simulink model "Sim2Real_variant_subsystem"  (R2025b)
settings: Solver=FixedStepDiscrete  StartTime=0.0  StopTime=inf  FixedStep=Ts_1ms  MaxStep=0.002  RelTol=1e-3
InitFcn:
  | modelFile = get_param(bdroot,'FileName');
  | if isempty(modelFile)
  |     error('The model must be saved before running InitFcn.');
  | end
  | 
  | % Folder where the .slx model is located
  | modelFolder = fileparts(char(modelFile));
  | 
  | % Find the parent folder named "resources" by going upwards
  | currentFolder  = modelFolder;
  | materialFolder = '';
  | 
  | while true
  |     [parentFolder, currentName] = fileparts(currentFolder);
  | 
  |     if strcmpi(currentName, 'resources')
  |         materialFolder = currentFolder;
  |         break;
  |     end
  | 
  |     if strcmp(parentFolder, currentFolder)
  |         error('Could not find a parent folder named "resources" starting from: %s', modelFolder);
  |     end
  | 
  |     currentFolder = parentFolder;
  | end
  | 
  | % Search recursively for the MuJoCo XML inside "material"
  | xmlSearch = dir(fullfile(materialFolder, '**', 'unitree_G1.xml'));
  | 
  | if isempty(xmlSearch)
  |     error('MuJoCo XML file not found inside material folder: %s', materialFolder);
  | elseif numel(xmlSearch) > 1
  |     error('Multiple unitree_G1.xml files found inside material folder. Leave only one valid XML.');
  | end
  | 
  | mujocoFolder = xmlSearch(1).folder;
  | xmlFullPath  = fullfile(xmlSearch(1).folder, xmlSearch(1).name);
  | 
  | % Save in base workspace in case you want to inspect them
  | assignin('base','modelFolder',modelFolder);
  | assignin('base','materialFolder',materialFolder);
  | assignin('base','mujocoFolder',mujocoFolder);
  | assignin('base','xmlFullPath',xmlFullPath);
  | 
  | % Final existence check
  | if exist(xmlFullPath,'file') ~= 2
  |     error('MuJoCo XML file not found: %s', xmlFullPath);
  | end
  | 
  | % Add the XML folder to the path so WHICH can find it
  | addpath(mujocoFolder, '-begin');
  | rehash path;
  | 
  | % Run launcher from the same folder as the model
  | launcherFile = fullfile(modelFolder, 'launcher.mlx');
  | if exist(launcherFile,'file') == 2
  |     run(launcherFile);
  | else
  |     error('Launcher file not found: %s', launcherFile);
  | end
  | 
  | % RUN_MODE:
  | if evalin('base', "exist('RUN_MODE','var')")
  |     tmp = evalin('base','RUN_MODE');
  |     if isa(tmp,'Simulink.Parameter')
  |         RUN_MODE = tmp;
  |     else
  |         RUN_MODE = Simulink.Parameter(tmp);
  |         RUN_MODE.CoderInfo.StorageClass = 'SimulinkGlobal';
  |         assignin('base','RUN_MODE',RUN_MODE);
  |     end
  | else
  |     RUN_MODE = Simulink.Parameter(0);
  |     RUN_MODE.CoderInfo.StorageClass = 'SimulinkGlobal';
  |     assignin('base','RUN_MODE',RUN_MODE);
  | end
StopFcn:
  | drawnow; pause(0.05);
  | 
  | % Stop figures
  | tags = {'G1_IMUState','G1_MotorState'};
  | for k = 1:numel(tags)
  |     delete(findall(0,'Type','uifigure','Tag',tags{k}));
  |     delete(findall(0,'Type','figure' , 'Tag',tags{k}));
  | end
undefined symbols (not defined in the file): crc, mode_machine, mode_pr, motor_cmd, reserve, Ts_1ms
libraries: ros2lib x3, mjLib x1
(part 1 of 2)
settings Model: Creator=vmano  LastModifiedBy=leffe
settings OptimizationCC: ReuseModelBlockBuffer=off
settings ModelReferenceCC: EnableRefExpFcnMdlSchedulingChecks=on
settings SFSimCC: SimTargetLang=C++  SimDLTargetLibrary=mkl-dnn
settings RTWCC: GPUComputeCapability=3.5

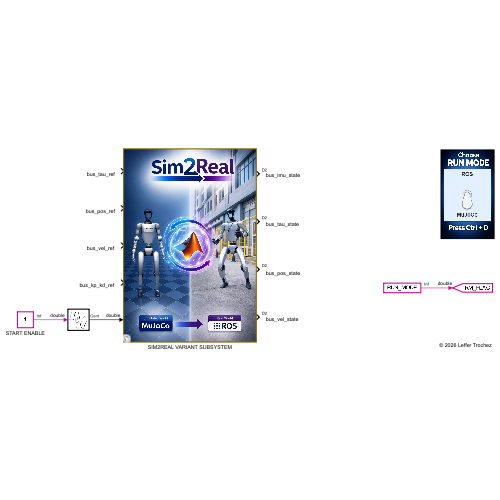
[thumbnail: Simulink's stored preview of the top-level diagram]
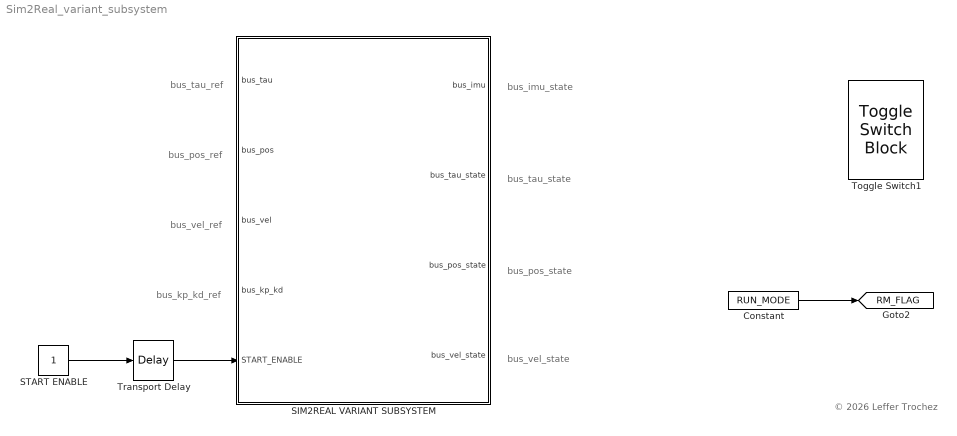
== system Sim2Real_variant_subsystem ==
  note: bus_tau_ref
  note: © 2026 Leffer Trochez
  note: bus_pos_ref
  note: bus_vel_ref
  note: bus_kp_kd_ref
  note: bus_imu_state
  note: bus_tau_state
  note: bus_pos_state
  note: bus_vel_state
  Constant : Constant  Value=RUN_MODE
  SIM2REAL VARIANT SUBSYSTEM : Subsystem  Variant=on  EmptyChoice=on
      mask Display: image('Sim2RealLogo2.png');
  START ENABLE : Constant
  Toggle Switch1 : ToggleSwitchBlock  LabelPosition=Hide
  Transport Delay : TransportDelay  DelayTime=2
  tag scope: RM_FLAG=global
  wires:
  START ENABLE/1 -> Transport Delay/1
  Constant/1 -> [RM_FLAG]
  Transport Delay/1 -> SIM2REAL VARIANT SUBSYSTEM/5(START_ENABLE)

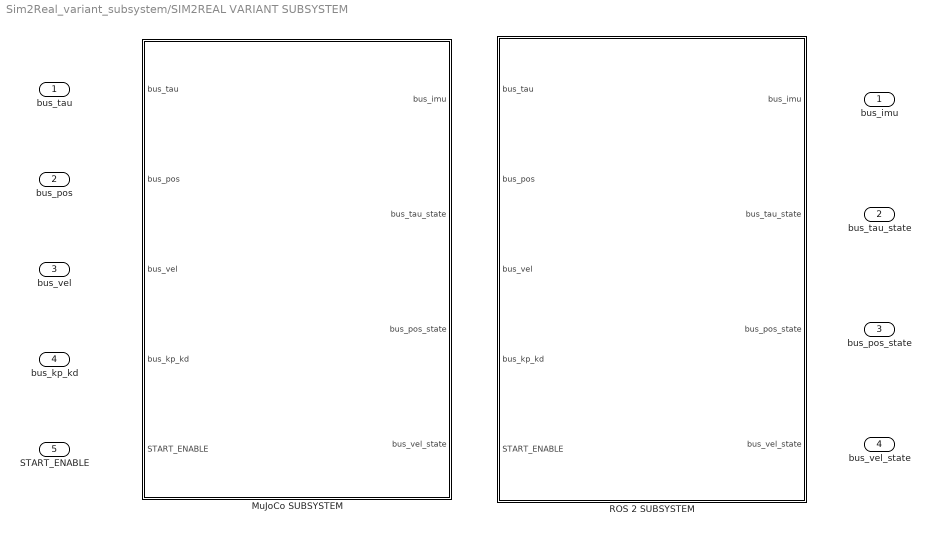
== system Sim2Real_variant_subsystem/SIM2REAL VARIANT SUBSYSTEM ==
  bus_tau : Inport  OutDataTypeStr=Bus: bus_tau_ref
  bus_pos : Inport  Port=2  OutDataTypeStr=Bus: bus_pos_ref
  bus_vel : Inport  Port=3  OutDataTypeStr=Bus: bus_vel_ref
  bus_kp_kd : Inport  Port=4  OutDataTypeStr=Bus: bus_kp_kd_dyn
  START_ENABLE : Inport  Port=5
  MuJoCo SUBSYSTEM : Subsystem  VariantControl=RUN_MODE == 0
      mask Display: image('MuJoCo G1.png');
  ROS 2 SUBSYSTEM : Subsystem  VariantControl=RUN_MODE == 1
      mask Display: image('Real G1.png');
  bus_imu : Outport  OutDataTypeStr=Bus: bus_imu
  bus_tau_state : Outport  Port=2  OutDataTypeStr=Bus: bus_tau_state
  bus_pos_state : Outport  Port=3  OutDataTypeStr=Bus: bus_pos_state
  bus_vel_state : Outport  Port=4  OutDataTypeStr=Bus: bus_vel_state

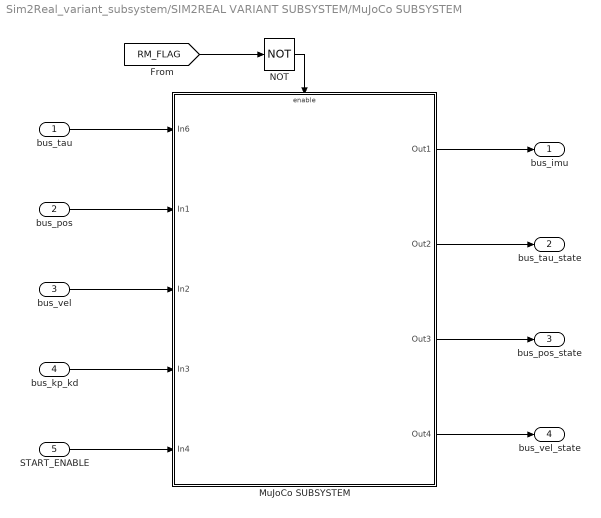
== system Sim2Real_variant_subsystem/SIM2REAL VARIANT SUBSYSTEM/MuJoCo SUBSYSTEM ==
  bus_tau : Inport  OutDataTypeStr=Bus: bus_tau_ref
  bus_pos : Inport  Port=2  OutDataTypeStr=Bus: bus_pos_ref
  bus_vel : Inport  Port=3  OutDataTypeStr=Bus: bus_vel_ref
  bus_kp_kd : Inport  Port=4  OutDataTypeStr=Bus: bus_kp_kd_dyn
  START_ENABLE : Inport  Port=5
  MuJoCo SUBSYSTEM : Subsystem  TreatAsAtomicUnit=on
      mask Display: image('MuJoCo G1.png');
  NOT : Logic  Operator=NOT  IconShape=distinctive  AllPortsSameDT=off  OutDataTypeStr=boolean
  bus_imu : Outport  OutDataTypeStr=Bus: bus_imu
  bus_tau_state : Outport  Port=2  OutDataTypeStr=Bus: bus_tau_state
  bus_pos_state : Outport  Port=3  OutDataTypeStr=Bus: bus_pos_state
  bus_vel_state : Outport  Port=4  OutDataTypeStr=Bus: bus_vel_state
  wires:
  [RM_FLAG] -> NOT/1
  NOT/1 -> MuJoCo SUBSYSTEM/Enable
  bus_tau/1 -> MuJoCo SUBSYSTEM/1(In6)
  bus_pos/1 -> MuJoCo SUBSYSTEM/2(In1)
  bus_vel/1 -> MuJoCo SUBSYSTEM/3(In2)
  bus_kp_kd/1 -> MuJoCo SUBSYSTEM/4(In3)
  START_ENABLE/1 -> MuJoCo SUBSYSTEM/5(In4)
  MuJoCo SUBSYSTEM/1(Out1) -> bus_imu/1
  MuJoCo SUBSYSTEM/2(Out2) -> bus_tau_state/1
  MuJoCo SUBSYSTEM/3(Out3) -> bus_pos_state/1
  MuJoCo SUBSYSTEM/4(Out4) -> bus_vel_state/1

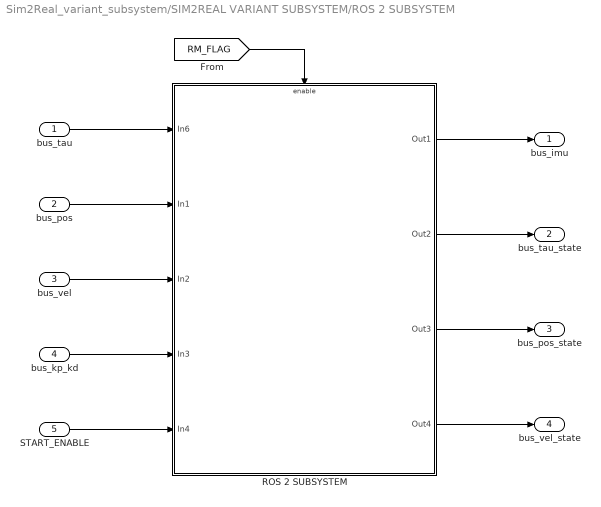
== system Sim2Real_variant_subsystem/SIM2REAL VARIANT SUBSYSTEM/ROS 2 SUBSYSTEM ==
  bus_tau : Inport  OutDataTypeStr=Bus: bus_tau_ref
  bus_pos : Inport  Port=2  OutDataTypeStr=Bus: bus_pos_ref
  bus_vel : Inport  Port=3  OutDataTypeStr=Bus: bus_vel_ref
  bus_kp_kd : Inport  Port=4  OutDataTypeStr=Bus: bus_kp_kd_dyn
  START_ENABLE : Inport  Port=5
  ROS 2 SUBSYSTEM : Subsystem  TreatAsAtomicUnit=on
      mask Display: image('Real G1.png');
  bus_imu : Outport  OutDataTypeStr=Bus: bus_imu
  bus_tau_state : Outport  Port=2  OutDataTypeStr=Bus: bus_tau_state
  bus_pos_state : Outport  Port=3  OutDataTypeStr=Bus: bus_pos_state
  bus_vel_state : Outport  Port=4  OutDataTypeStr=Bus: bus_vel_state
  wires:
  bus_tau/1 -> ROS 2 SUBSYSTEM/1(In6)
  bus_kp_kd/1 -> ROS 2 SUBSYSTEM/4(In3)
  bus_vel/1 -> ROS 2 SUBSYSTEM/3(In2)
  START_ENABLE/1 -> ROS 2 SUBSYSTEM/5(In4)
  bus_pos/1 -> ROS 2 SUBSYSTEM/2(In1)
  ROS 2 SUBSYSTEM/3(Out3) -> bus_pos_state/1
  ROS 2 SUBSYSTEM/2(Out2) -> bus_tau_state/1
  ROS 2 SUBSYSTEM/1(Out1) -> bus_imu/1
  ROS 2 SUBSYSTEM/4(Out4) -> bus_vel_state/1
  [RM_FLAG] -> ROS 2 SUBSYSTEM/Enable

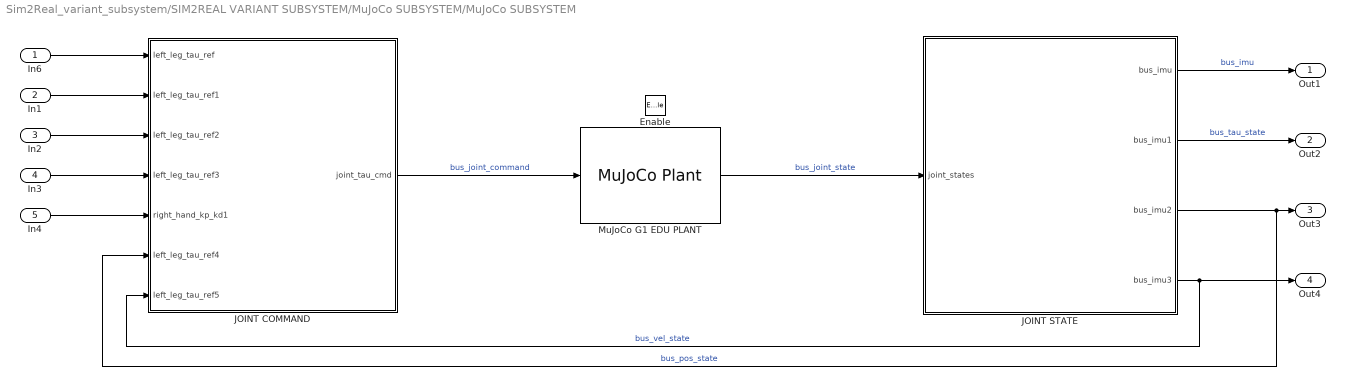
== system Sim2Real_variant_subsystem/SIM2REAL VARIANT SUBSYSTEM/MuJoCo SUBSYSTEM/MuJoCo SUBSYSTEM ==
  In6 : Inport  OutDataTypeStr=Bus: bus_tau_ref
  In1 : Inport  Port=2  OutDataTypeStr=Bus: bus_pos_ref
  In2 : Inport  Port=3  OutDataTypeStr=Bus: bus_vel_ref
  In3 : Inport  Port=4  OutDataTypeStr=Bus: bus_kp_kd_dyn
  In4 : Inport  Port=5
  Enable : EnablePort
  JOINT COMMAND : Subsystem
      mask Display: image('1.png');
  JOINT STATE : Subsystem
      mask Display: image('2.png');
  MuJoCo G1 EDU PLANT : mjLib/MuJoCo Plant  controlBus=[]  sensorBus=mj_bus_sensor_7979902499018342666  controlLength=[]  sensorLength=[]  rgbLength=[]  depthLength=[]  sampleTime=0.002  xmlFileRel=unitree_G1.xml  xmlFile=C:\Users\leffe\OneDrive - Universidad de los andes\GIAP research group\Conferences\ICRA 2026 - poster Sim2Real G1\resources\MuJoCo files\unitree_G1.xml  renderingType=Global  vsync=off  visualFPS=FPS_MuJoCo  zoomLevel=1  znear=0.032  zfar=160  cameraSampleTime=Ts_1ms  rgbOutOption=on  depthOutOption=off  controlInterfaceType=Bus
      settings: SourceProductName=MuJoCo Simulator
  Out1 : Outport  OutDataTypeStr=Bus: bus_imu
  Out2 : Outport  Port=2  OutDataTypeStr=Bus: bus_tau_state
  Out3 : Outport  Port=3  OutDataTypeStr=Bus: bus_pos_state
  Out4 : Outport  Port=4  OutDataTypeStr=Bus: bus_vel_state
  wires:
  JOINT COMMAND/1(joint_tau_cmd) -> MuJoCo G1 EDU PLANT/1  "bus_joint_command"
  MuJoCo G1 EDU PLANT/1 -> JOINT STATE/1(joint_states)  "bus_joint_state"
  In6/1 -> JOINT COMMAND/1(left_leg_tau_ref)
  In1/1 -> JOINT COMMAND/2(left_leg_tau_ref1)
  In2/1 -> JOINT COMMAND/3(left_leg_tau_ref2)
  In3/1 -> JOINT COMMAND/4(left_leg_tau_ref3)
  In4/1 -> JOINT COMMAND/5(right_hand_kp_kd1)
  JOINT STATE/2(bus_imu1) -> Out2/1  "bus_tau_state"
  JOINT STATE/3(bus_imu2) -> JOINT COMMAND/6(left_leg_tau_ref4), Out3/1  "bus_pos_state"
  JOINT STATE/4(bus_imu3) -> Out4/1, JOINT COMMAND/7(left_leg_tau_ref5)  "bus_vel_state"
  JOINT STATE/1(bus_imu) -> Out1/1  "bus_imu"

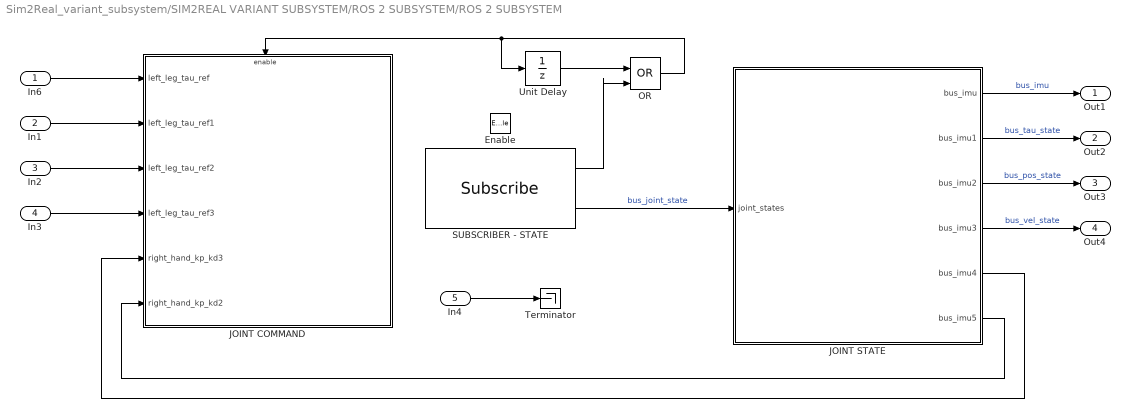
== system Sim2Real_variant_subsystem/SIM2REAL VARIANT SUBSYSTEM/ROS 2 SUBSYSTEM/ROS 2 SUBSYSTEM ==
  In6 : Inport  OutDataTypeStr=Bus: bus_tau_ref
  In1 : Inport  Port=2  OutDataTypeStr=Bus: bus_pos_ref
  In2 : Inport  Port=3  OutDataTypeStr=Bus: bus_vel_ref
  In3 : Inport  Port=4  OutDataTypeStr=Bus: bus_kp_kd_dyn
  In4 : Inport  Port=5
  Enable : EnablePort
  JOINT COMMAND : Subsystem  TreatAsAtomicUnit=on
      mask Display: image('8.png');
  JOINT STATE : Subsystem
      mask Display: image('9.png');
  OR : Logic  Operator=OR  IconShape=distinctive  AllPortsSameDT=off  OutDataTypeStr=boolean
  SUBSCRIBER - STATE : ros2lib/Subscribe  topicSource=Specify your own  topic=/lowstate  messageType=unitree_hg/LowState  sampleTime=Ts_1ms  QOSHistory=Keep last  QOSDepth=10  QOSReliability=Reliable  QOSDurability=Volatile  QOSDeadline=Inf  QOSLifespan=Inf  QOSLiveliness=Automatic  QOSLeaseDuration=Inf  QOSAvoidROSNamespaceConventions=off
  Terminator : Terminator
  Unit Delay : UnitDelay  SampleTime=0.002  HasFrameUpgradeWarning=on
  Out1 : Outport  OutDataTypeStr=Bus: bus_imu
  Out2 : Outport  Port=2  OutDataTypeStr=Bus: bus_tau_state
  Out3 : Outport  Port=3  OutDataTypeStr=Bus: bus_pos_state
  Out4 : Outport  Port=4  OutDataTypeStr=Bus: bus_vel_state
  wires:
  SUBSCRIBER - STATE/2 -> JOINT STATE/1(joint_states)  "bus_joint_state"
  SUBSCRIBER - STATE/1 -> OR/2
  OR/1 -> JOINT COMMAND/Enable, Unit Delay/1
  Unit Delay/1 -> OR/1
  JOINT STATE/6(bus_imu5) -> JOINT COMMAND/6(right_hand_kp_kd2)
  In2/1 -> JOINT COMMAND/3(left_leg_tau_ref2)
  In3/1 -> JOINT COMMAND/4(left_leg_tau_ref3)
  In4/1 -> Terminator/1
  In1/1 -> JOINT COMMAND/2(left_leg_tau_ref1)
  In6/1 -> JOINT COMMAND/1(left_leg_tau_ref)
  JOINT STATE/4(bus_imu3) -> Out4/1  "bus_vel_state"
  JOINT STATE/3(bus_imu2) -> Out3/1  "bus_pos_state"
  JOINT STATE/2(bus_imu1) -> Out2/1  "bus_tau_state"
  JOINT STATE/1(bus_imu) -> Out1/1  "bus_imu"
  JOINT STATE/5(bus_imu4) -> JOINT COMMAND/5(right_hand_kp_kd3)

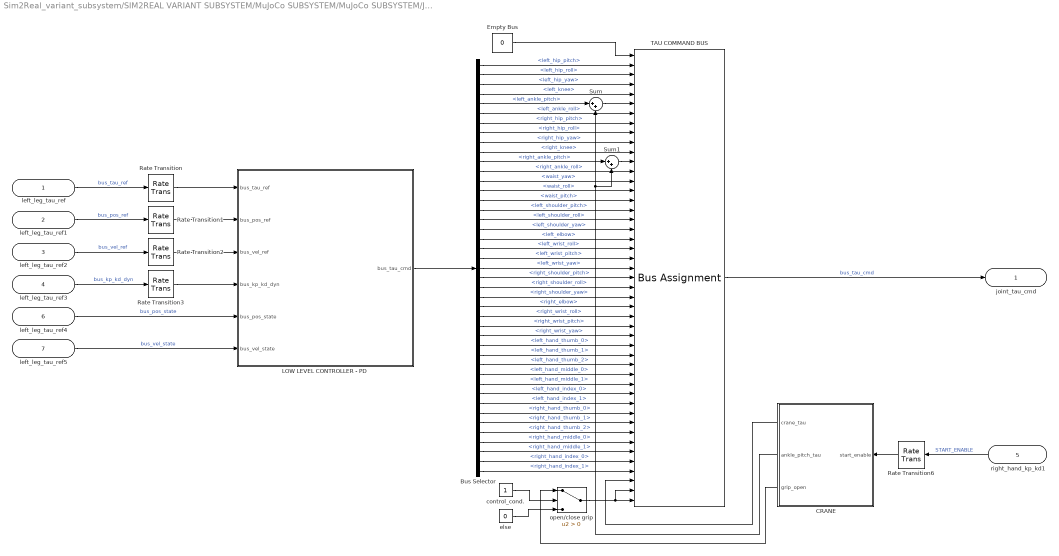
== system Sim2Real_variant_subsystem/SIM2REAL VARIANT SUBSYSTEM/MuJoCo SUBSYSTEM/MuJoCo SUBSYSTEM/JOINT COMMAND ==
  left_leg_tau_ref : Inport  OutDataTypeStr=Bus: bus_tau_ref
  left_leg_tau_ref1 : Inport  Port=2  OutDataTypeStr=Bus: bus_pos_ref
  left_leg_tau_ref2 : Inport  Port=3  OutDataTypeStr=Bus: bus_vel_ref
  left_leg_tau_ref3 : Inport  Port=4  OutDataTypeStr=Bus: bus_kp_kd_dyn
  right_hand_kp_kd1 : Inport  Port=5
  left_leg_tau_ref4 : Inport  Port=6  OutDataTypeStr=Bus: bus_pos_state
  left_leg_tau_ref5 : Inport  Port=7  OutDataTypeStr=Bus: bus_vel_state
  Bus Selector : BusSelector  OutputSignals=left_hip_pitch,left_hip_roll,left_hip_yaw,left_knee,left_ankle_pitch,left_ankle_roll,right_hip_pitch,right_hip_roll,right_hip_yaw,right_knee,right_ankle_pitch,right_ankle_roll,waist_yaw,waist_roll,waist_pitch,left_shoulder_pitch,left_shoulder_roll,left_shoulder_yaw,left_elbow,left_wrist_roll,left_wrist_pitch,left_wrist_yaw,right_shoulder_pitch,right_shoulder_roll,right_shoulder_yaw,right_elbow,right_wrist_roll,right_wrist_pitch,right_wrist_yaw,left_hand_thumb_0,left_hand_thumb_1,left_hand_thumb_2,left_hand_middle_0,left_hand_middle_1,left_hand_index_0,left_hand_index_1,right_hand_thumb_0,right_hand_thumb_1,right_hand_thumb_2,right_hand_middle_0,right_hand_middle_1,right_hand_index_0,right_hand_index_1
  CRANE : MATLAB Function  TreatAsAtomicUnit=on
  Empty Bus : Constant  Value=0  OutDataTypeStr=Bus: mj_bus_input_303657145477151593  LockScale=on
  LOW LEVEL CONTROLLER - PD : MATLAB Function  TreatAsAtomicUnit=on
  Rate Transition{,1..3,6} (5 alike) : RateTransition  OutPortSampleTime=Ts_1ms
  Sum : Sum  Inputs=|++
  Sum1 : Sum  Inputs=|++
  TAU COMMAND BUS : BusAssignment  AssignedSignals=left_hip_pitch,left_hip_roll,left_hip_yaw,left_knee,left_ankle_pitch,left_ankle_roll,right_hip_pitch,right_hip_roll,right_hip_yaw,right_knee,right_ankle_pitch,right_ankle_roll,waist_yaw,waist_roll,waist_pitch,left_shoulder_pitch,left_shoulder_roll,left_shoulder_yaw,left_elbow,left_wrist_roll,left_wrist_pitch,left_wrist_yaw,right_shoulder_pitch,right_shoulder_roll,right_shoulder_yaw,right_elbow,right_wrist_roll,right_wrist_pitch,right_wrist_yaw,left_hand_thumb_0,left_hand_thumb_1,left_hand_thumb_2,left_hand_middle_0,left_hand_middle_1,left_hand_index_0,left_hand_index_1,right_hand_thumb_0,right_hand_thumb_1,right_hand_thumb_2,right_hand_middle_0,right_hand_middle_1,right_hand_index_0,right_hand_index_1,crane_tau,grip_open_R,grip_open_L
  control_cond. : Constant
  else : Constant  Value=0
  open/close grip : Switch  Criteria=u2 > Threshold  SaturateOnIntegerOverflow=off  InputSameDT=off
  joint_tau_cmd : Outport  OutDataTypeStr=Bus: mj_bus_input_303657145477151593
  wires:
  Sum1/1 -> TAU COMMAND BUS/12
  Empty Bus/1 -> TAU COMMAND BUS/1
  CRANE/2(ankle_pitch_tau) -> Sum1/2, Sum/2
  Sum/1 -> TAU COMMAND BUS/6
  CRANE/3(grip_open) -> open/close grip/1
  right_hand_kp_kd1/1 -> Rate Transition6/1  "START_ENABLE"
  TAU COMMAND BUS/1 -> joint_tau_cmd/1  "bus_tau_cmd"
  left_leg_tau_ref/1 -> Rate Transition/1  "bus_tau_ref"
  left_leg_tau_ref1/1 -> Rate Transition1/1  "bus_pos_ref"
  left_leg_tau_ref2/1 -> Rate Transition2/1  "bus_vel_ref"
  left_leg_tau_ref3/1 -> Rate Transition3/1  "bus_kp_kd_dyn"
  left_leg_tau_ref4/1 -> LOW LEVEL CONTROLLER - PD/5(bus_pos_state)  "bus_pos_state"
  left_leg_tau_ref5/1 -> LOW LEVEL CONTROLLER - PD/6(bus_vel_state)  "bus_vel_state"
  CRANE/1(crane_tau) -> TAU COMMAND BUS/45
  Rate Transition/1 -> LOW LEVEL CONTROLLER - PD/1(bus_tau_ref)
  Rate Transition1/1 -> LOW LEVEL CONTROLLER - PD/2(bus_pos_ref)
  Rate Transition2/1 -> LOW LEVEL CONTROLLER - PD/3(bus_vel_ref)
  Rate Transition3/1 -> LOW LEVEL CONTROLLER - PD/4(bus_kp_kd_dyn)
  Rate Transition6/1 -> CRANE/1(start_enable)
  LOW LEVEL CONTROLLER - PD/1(bus_tau_cmd) -> Bus Selector/1
  Bus Selector/11 -> Sum1/1  "<right_ankle_pitch>"
  Bus Selector/5 -> Sum/1  "<left_ankle_pitch>"
  Bus Selector/1 -> TAU COMMAND BUS/2  "<left_hip_pitch>"
  Bus Selector/2 -> TAU COMMAND BUS/3  "<left_hip_roll>"
  Bus Selector/3 -> TAU COMMAND BUS/4  "<left_hip_yaw>"
  Bus Selector/4 -> TAU COMMAND BUS/5  "<left_knee>"
  Bus Selector/6 -> TAU COMMAND BUS/7  "<left_ankle_roll>"
  Bus Selector/7 -> TAU COMMAND BUS/8  "<right_hip_pitch>"
  Bus Selector/8 -> TAU COMMAND BUS/9  "<right_hip_roll>"
  Bus Selector/9 -> TAU COMMAND BUS/10  "<right_hip_yaw>"
  Bus Selector/10 -> TAU COMMAND BUS/11  "<right_knee>"
  Bus Selector/12 -> TAU COMMAND BUS/13  "<right_ankle_roll>"
  Bus Selector/13 -> TAU COMMAND BUS/14  "<waist_yaw>"
  Bus Selector/14 -> TAU COMMAND BUS/15  "<waist_roll>"
  Bus Selector/15 -> TAU COMMAND BUS/16  "<waist_pitch>"
  Bus Selector/16 -> TAU COMMAND BUS/17  "<left_shoulder_pitch>"
  Bus Selector/17 -> TAU COMMAND BUS/18  "<left_shoulder_roll>"
  Bus Selector/18 -> TAU COMMAND BUS/19  "<left_shoulder_yaw>"
  Bus Selector/19 -> TAU COMMAND BUS/20  "<left_elbow>"
  Bus Selector/20 -> TAU COMMAND BUS/21  "<left_wrist_roll>"
  Bus Selector/21 -> TAU COMMAND BUS/22  "<left_wrist_pitch>"
  Bus Selector/22 -> TAU COMMAND BUS/23  "<left_wrist_yaw>"
  Bus Selector/23 -> TAU COMMAND BUS/24  "<right_shoulder_pitch>"
  Bus Selector/24 -> TAU COMMAND BUS/25  "<right_shoulder_roll>"
  Bus Selector/25 -> TAU COMMAND BUS/26  "<right_shoulder_yaw>"
  Bus Selector/26 -> TAU COMMAND BUS/27  "<right_elbow>"
  Bus Selector/27 -> TAU COMMAND BUS/28  "<right_wrist_roll>"
  Bus Selector/28 -> TAU COMMAND BUS/29  "<right_wrist_pitch>"
  Bus Selector/29 -> TAU COMMAND BUS/30  "<right_wrist_yaw>"
  Bus Selector/30 -> TAU COMMAND BUS/31  "<left_hand_thumb_0>"
  Bus Selector/31 -> TAU COMMAND BUS/32  "<left_hand_thumb_1>"
  Bus Selector/32 -> TAU COMMAND BUS/33  "<left_hand_thumb_2>"
  Bus Selector/33 -> TAU COMMAND BUS/34  "<left_hand_middle_0>"
  Bus Selector/34 -> TAU COMMAND BUS/35  "<left_hand_middle_1>"
  Bus Selector/35 -> TAU COMMAND BUS/36  "<left_hand_index_0>"
  Bus Selector/36 -> TAU COMMAND BUS/37  "<left_hand_index_1>"
  Bus Selector/37 -> TAU COMMAND BUS/38  "<right_hand_thumb_0>"
  Bus Selector/38 -> TAU COMMAND BUS/39  "<right_hand_thumb_1>"
  Bus Selector/39 -> TAU COMMAND BUS/40  "<right_hand_thumb_2>"
  Bus Selector/40 -> TAU COMMAND BUS/41  "<right_hand_middle_0>"
  Bus Selector/41 -> TAU COMMAND BUS/42  "<right_hand_middle_1>"
  Bus Selector/42 -> TAU COMMAND BUS/43  "<right_hand_index_0>"
  Bus Selector/43 -> TAU COMMAND BUS/44  "<right_hand_index_1>"
  control_cond./1 -> open/close grip/2
  else/1 -> open/close grip/3
  open/close grip/1 -> TAU COMMAND BUS/47, TAU COMMAND BUS/46

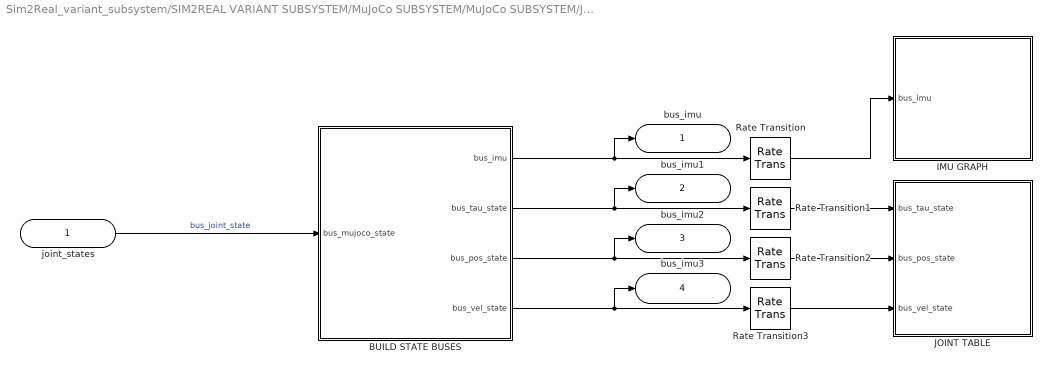
== system Sim2Real_variant_subsystem/SIM2REAL VARIANT SUBSYSTEM/MuJoCo SUBSYSTEM/MuJoCo SUBSYSTEM/JOINT STATE ==
  joint_states : Inport  OutDataTypeStr=Bus: mj_bus_sensor_13323796724550544295
  BUILD STATE BUSES : MATLAB Function  TreatAsAtomicUnit=on
  IMU GRAPH : MATLAB Function  TreatAsAtomicUnit=on
  JOINT TABLE : MATLAB Function  TreatAsAtomicUnit=on
  Rate Transition{,1..3} (4 alike) : RateTransition  OutPortSampleTime=Ts_UIs
  bus_imu : Outport  OutDataTypeStr=Bus: bus_imu
  bus_imu1 : Outport  Port=2  OutDataTypeStr=Bus: bus_tau_state
  bus_imu2 : Outport  Port=3  OutDataTypeStr=Bus: bus_pos_state
  bus_imu3 : Outport  Port=4  OutDataTypeStr=Bus: bus_vel_state
  wires:
  joint_states/1 -> BUILD STATE BUSES/1(bus_mujoco_state)  "bus_joint_state"
  BUILD STATE BUSES/1(bus_imu) -> Rate Transition/1, bus_imu/1
  BUILD STATE BUSES/3(bus_pos_state) -> Rate Transition2/1, bus_imu2/1
  BUILD STATE BUSES/2(bus_tau_state) -> Rate Transition1/1, bus_imu1/1
  BUILD STATE BUSES/4(bus_vel_state) -> Rate Transition3/1, bus_imu3/1
  Rate Transition/1 -> IMU GRAPH/1(bus_imu)
  Rate Transition1/1 -> JOINT TABLE/1(bus_tau_state)
  Rate Transition2/1 -> JOINT TABLE/2(bus_pos_state)
  Rate Transition3/1 -> JOINT TABLE/3(bus_vel_state)

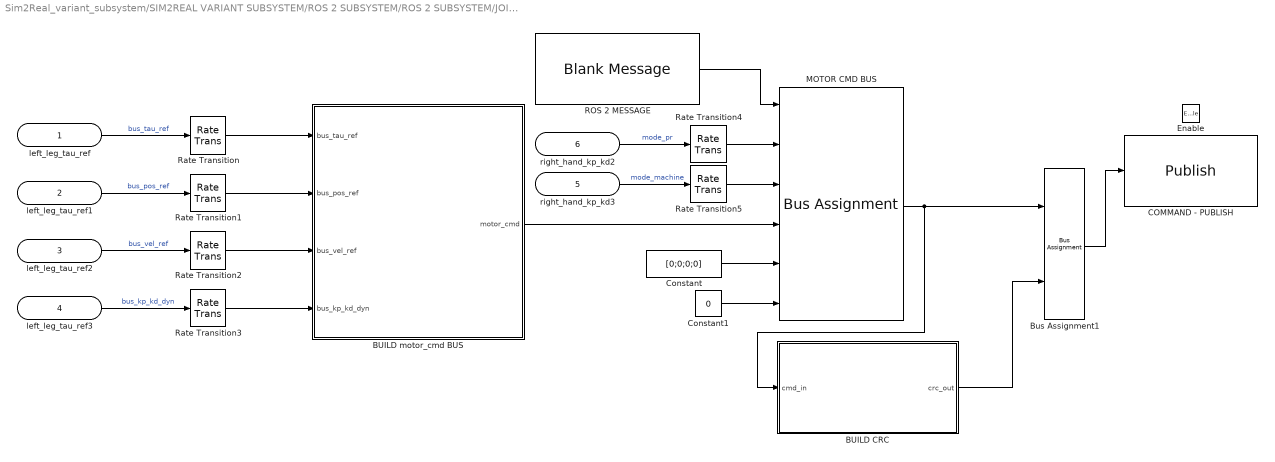
== system Sim2Real_variant_subsystem/SIM2REAL VARIANT SUBSYSTEM/ROS 2 SUBSYSTEM/ROS 2 SUBSYSTEM/JOINT COMMAND ==
  left_leg_tau_ref : Inport  OutDataTypeStr=Bus: bus_tau_ref
  left_leg_tau_ref1 : Inport  Port=2  OutDataTypeStr=Bus: bus_pos_ref
  left_leg_tau_ref2 : Inport  Port=3  OutDataTypeStr=Bus: bus_vel_ref
  left_leg_tau_ref3 : Inport  Port=4  OutDataTypeStr=Bus: bus_kp_kd_dyn
  right_hand_kp_kd3 : Inport  Port=5
  right_hand_kp_kd2 : Inport  Port=6
  Enable : EnablePort
  BUILD CRC : MATLAB Function  TreatAsAtomicUnit=on
  BUILD motor_cmd BUS : MATLAB Function  TreatAsAtomicUnit=on
  Bus Assignment1 : BusAssignment  AssignedSignals=crc
  COMMAND - PUBLISH : ros2lib/Publish  topicSource=Specify your own  topic=/lowcmd  messageType=unitree_hg/LowCmd  QOSHistory=Keep last  QOSDepth=10  QOSReliability=Reliable  QOSDurability=Volatile  QOSDeadline=Inf  QOSLifespan=Inf  QOSLiveliness=Automatic  QOSLeaseDuration=Inf  QOSAvoidROSNamespaceConventions=off
  Constant : Constant  Value=[0;0;0;0]  OutDataTypeStr=uint32
  Constant1 : Constant  Value=0  OutDataTypeStr=uint32
  MOTOR CMD BUS : BusAssignment  AssignedSignals=mode_pr,mode_machine,motor_cmd,reserve,crc
  ROS 2 MESSAGE : ros2lib/Blank Message  messageClass=Message  entityType=unitree_hg/LowCmd  messageType=unitree_hg/LowCmd  SampleTime=Ts_1ms
  Rate Transition{,1..5} (6 alike) : RateTransition  OutPortSampleTime=Ts_1ms
  wires:
  right_hand_kp_kd3/1 -> Rate Transition5/1  "mode_machine"
  left_leg_tau_ref/1 -> Rate Transition/1  "bus_tau_ref"
  right_hand_kp_kd2/1 -> Rate Transition4/1  "mode_pr"
  ROS 2 MESSAGE/1 -> MOTOR CMD BUS/1
  BUILD motor_cmd BUS/1(motor_cmd) -> MOTOR CMD BUS/4
  MOTOR CMD BUS/1 -> BUILD CRC/1(cmd_in), Bus Assignment1/1
  BUILD CRC/1(crc_out) -> Bus Assignment1/2
  Constant/1 -> MOTOR CMD BUS/5
  Constant1/1 -> MOTOR CMD BUS/6
  Bus Assignment1/1 -> COMMAND - PUBLISH/1
  left_leg_tau_ref1/1 -> Rate Transition1/1  "bus_pos_ref"
  left_leg_tau_ref2/1 -> Rate Transition2/1  "bus_vel_ref"
  left_leg_tau_ref3/1 -> Rate Transition3/1  "bus_kp_kd_dyn"
  Rate Transition/1 -> BUILD motor_cmd BUS/1(bus_tau_ref)
  Rate Transition1/1 -> BUILD motor_cmd BUS/2(bus_pos_ref)
  Rate Transition2/1 -> BUILD motor_cmd BUS/3(bus_vel_ref)
  Rate Transition3/1 -> BUILD motor_cmd BUS/4(bus_kp_kd_dyn)
  Rate Transition4/1 -> MOTOR CMD BUS/2
  Rate Transition5/1 -> MOTOR CMD BUS/3

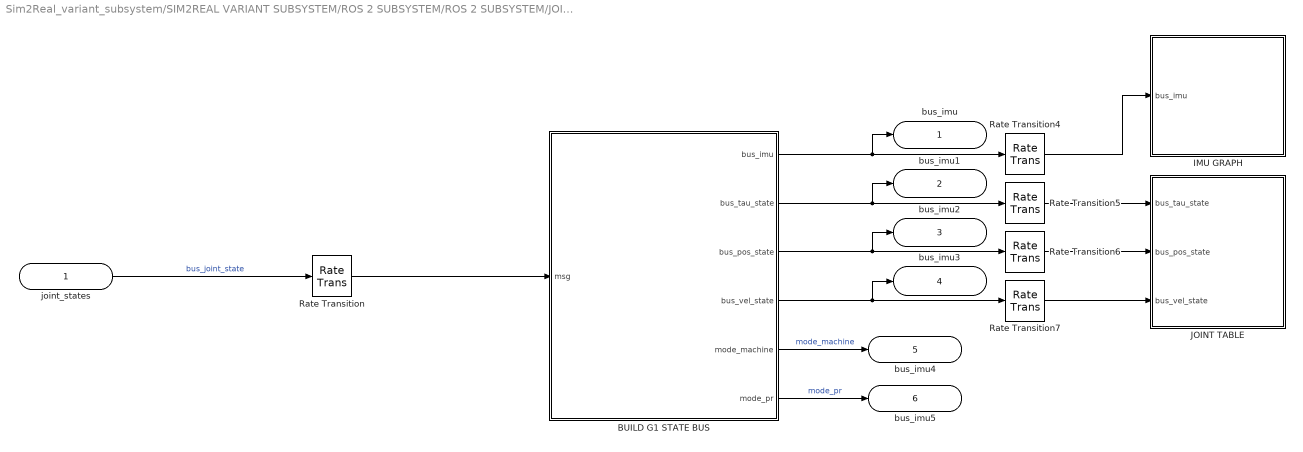
== system Sim2Real_variant_subsystem/SIM2REAL VARIANT SUBSYSTEM/ROS 2 SUBSYSTEM/ROS 2 SUBSYSTEM/JOINT STATE ==
  joint_states : Inport
  BUILD G1 STATE BUS : MATLAB Function  TreatAsAtomicUnit=on
  IMU GRAPH : MATLAB Function  TreatAsAtomicUnit=on
  JOINT TABLE : MATLAB Function  TreatAsAtomicUnit=on
  Rate Transition : RateTransition  OutPortSampleTime=0.002
  Rate Transition{4..7} (4 alike) : RateTransition  OutPortSampleTime=Ts_UIs
  bus_imu : Outport  OutDataTypeStr=Bus: bus_imu
  bus_imu1 : Outport  Port=2  OutDataTypeStr=Bus: bus_tau_state
  bus_imu2 : Outport  Port=3  OutDataTypeStr=Bus: bus_pos_state
  bus_imu3 : Outport  Port=4  OutDataTypeStr=Bus: bus_vel_state
  bus_imu4 : Outport  Port=5
  bus_imu5 : Outport  Port=6
  wires:
  joint_states/1 -> Rate Transition/1  "bus_joint_state"
  BUILD G1 STATE BUS/5(mode_machine) -> bus_imu4/1  "mode_machine"
  BUILD G1 STATE BUS/6(mode_pr) -> bus_imu5/1  "mode_pr"
  Rate Transition5/1 -> JOINT TABLE/1(bus_tau_state)
  Rate Transition6/1 -> JOINT TABLE/2(bus_pos_state)
  BUILD G1 STATE BUS/3(bus_pos_state) -> bus_imu2/1, Rate Transition6/1
  BUILD G1 STATE BUS/2(bus_tau_state) -> bus_imu1/1, Rate Transition5/1
  Rate Transition4/1 -> IMU GRAPH/1(bus_imu)
  BUILD G1 STATE BUS/1(bus_imu) -> bus_imu/1, Rate Transition4/1
  BUILD G1 STATE BUS/4(bus_vel_state) -> bus_imu3/1, Rate Transition7/1
  Rate Transition7/1 -> JOINT TABLE/3(bus_vel_state)
  Rate Transition/1 -> BUILD G1 STATE BUS/1(msg)

== matlab function Sim2Real_variant_subsystem/SIM2REAL VARIANT SUBSYSTEM/MuJoCo SUBSYSTEM/MuJoCo SUBSYSTEM/JOINT COMMAND/LOW LEVEL CONTROLLER - PD ==
  data: bus_tau_cmd output Bus: bus_tau_cmd; bus_tau_ref input Bus: bus_tau_ref; bus_pos_ref input Bus: bus_pos_ref; bus_vel_ref input Bus: bus_vel_ref; bus_kp_kd_dyn input Bus: bus_kp_kd_dyn; bus_pos_state input Bus: bus_pos_state; bus_vel_state input Bus: bus_vel_state; P_G1_CONSTRAINTS parameter
 function bus_tau_cmd = low_level_pd_controller_function( ...
    bus_tau_ref, bus_pos_ref, bus_vel_ref, bus_kp_kd_dyn, ...
    bus_pos_state, bus_vel_state, P_G1_CONSTRAINTS)
%#codegen

% Default output bus
bus_tau_cmd = struct( ...
    'left_hip_pitch',      0, ...
    'left_hip_roll',       0, ...
    'left_hip_yaw',        0, ...
    'left_knee',           0, ...
    'left_ankle_pitch',    0, ...
    'left_ankle_roll',     0, ...
    'right_hip_pitch',     0, ...
    'right_hip_roll',      0, ...
    'right_hip_yaw',       0, ...
    'right_knee',          0, ...
    'right_ankle_pitch',   0, ...
    'right_ankle_roll',    0, ...
    'waist_yaw',           0, ...
    'waist_roll',          0, ...
    'waist_pitch',         0, ...
    'left_shoulder_pitch', 0, ...
    'left_shoulder_roll',  0, ...
    'left_shoulder_yaw',   0, ...
    'left_elbow',          0, ...
    'left_wrist_roll',     0, ...
    'left_wrist_pitch',    0, ...
    'left_wrist_yaw',      0, ...
    'right_shoulder_pitch',0, ...
    'right_shoulder_roll', 0, ...
    'right_shoulder_yaw',  0, ...
    'right_elbow',         0, ...
    'right_wrist_roll',    0, ...
    'right_wrist_pitch',   0, ...
    'right_wrist_yaw',     0, ...
    'left_hand_thumb_0',   0, ...
    'left_hand_thumb_1',   0, ...
    'left_hand_thumb_2',   0, ...
    'left_hand_middle_0',  0, ...
    'left_hand_middle_1',  0, ...
    'left_hand_index_0',   0, ...
    'left_hand_index_1',   0, ...
    'right_hand_thumb_0',  0, ...
    'right_hand_thumb_1',  0, ...
    'right_hand_thumb_2',  0, ...
    'right_hand_middle_0', 0, ...
    'right_hand_middle_1', 0, ...
    'right_hand_index_0',  0, ...
    'right_hand_index_1',  0);

% Unpack reference buses

% tau refs
left_leg_tau_ref   = bus_tau_ref.left_leg_tau_ref;
right_leg_tau_ref  = bus_tau_ref.right_leg_tau_ref;
waist_tau_ref      = bus_tau_ref.waist_tau_ref;
left_arm_tau_ref   = bus_tau_ref.left_arm_tau_ref;
right_arm_tau_ref  = bus_tau_ref.right_arm_tau_ref;

% pos refs
left_leg_pos_ref   = bus_pos_ref.left_leg_pos_ref;
right_leg_pos_ref  = bus_pos_ref.right_leg_pos_ref;
waist_pos_ref      = bus_pos_ref.waist_pos_ref;
left_arm_pos_ref   = bus_pos_ref.left_arm_pos_ref;
right_arm_pos_ref  = bus_pos_ref.right_arm_pos_ref;

% vel refs
left_leg_vel_ref   = bus_vel_ref.left_leg_vel_ref;
right_leg_vel_ref  = bus_vel_ref.right_leg_vel_ref;
waist_vel_ref      = bus_vel_ref.waist_vel_ref;
left_arm_vel_ref   = bus_vel_ref.left_arm_vel_ref;
right_arm_vel_ref  = bus_vel_ref.right_arm_vel_ref;

% dynamic gains
left_leg_kp_kd   = bus_kp_kd_dyn.left_leg_kp_kd_dyn;
right_leg_kp_kd  = bus_kp_kd_dyn.right_leg_kp_kd_dyn;
waist_kp_kd      = bus_kp_kd_dyn.waist_kp_kd_dyn;
left_arm_kp_kd   = bus_kp_kd_dyn.left_arm_kp_kd_dyn;
right_arm_kp_kd  = bus_kp_kd_dyn.right_arm_kp_kd_dyn;

% Unpack state buses

% measured positions
left_leg_pos_state   = bus_pos_state.left_leg_pos_state;
right_leg_pos_state  = bus_pos_state.right_leg_pos_state;
waist_pos_state      = bus_pos_state.waist_pos_state;
left_arm_pos_state   = bus_pos_state.left_arm_pos_state;
right_arm_pos_state  = bus_pos_state.right_arm_pos_state;

% measured velocities
left_leg_vel_state   = bus_vel_state.left_leg_vel_state;
right_leg_vel_state  = bus_vel_state.right_leg_vel_state;
waist_vel_state      = bus_vel_state.waist_vel_state;
left_arm_vel_state   = bus_vel_state.left_arm_vel_state;
right_arm_vel_state  = bus_vel_state.right_arm_vel_state;

% Split Kp / Kd

Kp_left_leg   = left_leg_kp_kd(:,1);
Kd_left_leg   = left_leg_kp_kd(:,2);

Kp_right_leg  = right_leg_kp_kd(:,1);
Kd_right_leg  = right_leg_kp_kd(:,2);

Kp_waist      = waist_kp_kd(:,1);
Kd_waist      = waist_kp_kd(:,2);

Kp_left_arm   = left_arm_kp_kd(:,1);
Kd_left_arm   = left_arm_kp_kd(:,2);

Kp_right_arm  = right_arm_kp_kd(:,1);
Kd_right_arm  = right_arm_kp_kd(:,2);

% Position and velocity errors

e_left_leg   = left_leg_pos_ref   - left_leg_pos_state;
de_left_leg  = left_leg_vel_ref   - left_leg_vel_state;

e_right_leg  = right_leg_pos_ref  - right_leg_pos_state;
de_right_leg = right_leg_vel_ref  - right_leg_vel_state;

e_waist      = waist_pos_ref      - waist_pos_state;
de_waist     = waist_vel_ref      - waist_vel_state;

e_left_arm   = left_arm_pos_ref   - left_arm_pos_state;
de_left_arm  = left_arm_vel_ref   - left_arm_vel_state;

e_right_arm  = right_arm_pos_ref  - right_arm_pos_state;
de_right_arm = right_arm_vel_ref  - right_arm_vel_state;

% PD + feedforward torque
left_leg_tau_cmd   = left_leg_tau_ref   + Kp_left_leg   .* e_left_leg   + Kd_left_leg   .* de_left_leg;
right_leg_tau_cmd  = right_leg_tau_ref  + Kp_right_leg  .* e_right_leg  + Kd_right_leg  .* de_right_leg;
waist_tau_cmd      = waist_tau_ref      + Kp_waist      .* e_waist      + Kd_waist      .* de_waist;
left_arm_tau_cmd   = left_arm_tau_ref   + Kp_left_arm   .* e_left_arm   + Kd_left_arm   .* de_left_arm;
right_arm_tau_cmd  = right_arm_tau_ref  + Kp_right_arm  .* e_right_arm  + Kd_right_arm  .* de_right_arm;

% Torque saturation using robot constraints

tau_abs = P_G1_CONSTRAINTS.tau_abs;

tau_abs_left_leg   = tau_abs(P_G1_CONSTRAINTS.idx_left_leg);
tau_abs_right_leg  = tau_abs(P_G1_CONSTRAINTS.idx_right_leg);
tau_abs_waist      = tau_abs(P_G1_CONSTRAINTS.idx_waist);
tau_abs_left_arm   = tau_abs(P_G1_CONSTRAINTS.idx_left_arm);
tau_abs_right_arm  = tau_abs(P_G1_CONSTRAINTS.idx_right_arm);

left_leg_tau_cmd   = min(max(left_leg_tau_cmd,   -tau_abs_left_leg),   tau_abs_left_leg);
right_leg_tau_cmd  = min(max(right_leg_tau_cmd,  -tau_abs_right_leg),  tau_abs_right_leg);
waist_tau_cmd      = min(max(waist_tau_cmd,      -tau_abs_waist),      tau_abs_waist);
left_arm_tau_cmd   = min(max(left_arm_tau_cmd,   -tau_abs_left_arm),   tau_abs_left_arm);
right_arm_tau_cmd  = min(max(right_arm_tau_cmd,  -tau_abs_right_arm),  tau_abs_right_arm);

% Pack final joint-ordered output bus

% left leg
bus_tau_cmd.left_hip_pitch    = left_leg_tau_cmd(1);
bus_tau_cmd.left_hip_roll     = left_leg_tau_cmd(2);
bus_tau_cmd.left_hip_yaw      = left_leg_tau_cmd(3);
bus_tau_cmd.left_knee         = left_leg_tau_cmd(4);
bus_tau_cmd.left_ankle_pitch  = left_leg_tau_cmd(5);
bus_tau_cmd.left_ankle_roll   = left_leg_tau_cmd(6);

% right leg
bus_tau_cmd.right_hip_pitch   = right_leg_tau_cmd(1);
bus_tau_cmd.right_hip_roll    = right_leg_tau_cmd(2);
bus_tau_cmd.right_hip_yaw     = right_leg_tau_cmd(3);
bus_tau_cmd.right_knee        = right_leg_tau_cmd(4);
bus_tau_cmd.right_ankle_pitch = right_leg_tau_cmd(5);
bus_tau_cmd.right_ankle_roll  = right_leg_tau_cmd(6);

% waist
bus_tau_cmd.waist_yaw         = waist_tau_cmd(1);
bus_tau_cmd.waist_roll        = waist_tau_cmd(2);
bus_tau_cmd.waist_pitch       = waist_tau_cmd(3);

% left arm
bus_tau_cmd.left_shoulder_pitch = left_arm_tau_cmd(1);
bus_tau_cmd.left_shoulder_roll  = left_arm_tau_cmd(2);
bus_tau_cmd.left_shoulder_yaw   = left_arm_tau_cmd(3);
bus_tau_cmd.left_elbow          = left_arm_tau_cmd(4);
bus_tau_cmd.left_wrist_roll     = left_arm_tau_cmd(5);
bus_tau_cmd.left_wrist_pitch    = left_arm_tau_cmd(6);
bus_tau_cmd.left_wrist_yaw      = left_arm_tau_cmd(7);

% right arm
bus_tau_cmd.right_shoulder_pitch = right_arm_tau_cmd(1);
bus_tau_cmd.right_shoulder_roll  = right_arm_tau_cmd(2);
bus_tau_cmd.right_shoulder_yaw   = right_arm_tau_cmd(3);
bus_tau_cmd.right_elbow          = right_arm_tau_cmd(4);
bus_tau_cmd.right_wrist_roll     = right_arm_tau_cmd(5);
bus_tau_cmd.right_wrist_pitch    = right_arm_tau_cmd(6);
bus_tau_cmd.right_wrist_yaw      = right_arm_tau_cmd(7);

% hands disabled for now
bus_tau_cmd.left_hand_thumb_0   = 0;
bus_tau_cmd.left_hand_thumb_1   = 0;
bus_tau_cmd.left_hand_thumb_2   = 0;
bus_tau_cmd.left_hand_middle_0  = 0;
bus_tau_cmd.left_hand_middle_1  = 0;
bus_tau_cmd.left_hand_index_0   = 0;
bus_tau_cmd.left_hand_index_1   = 0;

bus_tau_cmd.right_hand_thumb_0  = 0;
bus_tau_cmd.right_hand_thumb_1  = 0;
bus_tau_cmd.right_hand_thumb_2  = 0;
bus_tau_cmd.right_hand_middle_0 = 0;
bus_tau_cmd.right_hand_middle_1 = 0;
bus_tau_cmd.right_hand_index_0  = 0;
bus_tau_cmd.right_hand_index_1  = 0;

end

== matlab function Sim2Real_variant_subsystem/SIM2REAL VARIANT SUBSYSTEM/MuJoCo SUBSYSTEM/MuJoCo SUBSYSTEM/JOINT STATE/IMU GRAPH ==
  settings: updateMethod=DISCRETE
  data: bus_imu input Bus: bus_imu; P_MACHINE_DATA parameter
function imu_graph_function(bus_imu, P_MACHINE_DATA)
%#codegen

coder.extrinsic('figure','subplot','plot3','line','legend','title', ...
                'grid','axis','xlim','ylim','zlim','view','hold','set', ...
                'drawnow','text','xlabel','ylabel');

persistent fig ax3 axA axG ...
           hX hY hZ ...
           la1 la2 la3 ...
           lg1 lg2 lg3 ...
           txtYPR ...
           Tbuf Abuf Gbuf ...
           Nbuf nsamp kbuf ...
           inited ...
           windowSec ...
           Ts_ui ...
           frame_count ...
           orient_div ...
           axis_div ...
           last_xlim_update

if ~(P_MACHINE_DATA.active_IMU_graph ~= 0)
    return;
end

Ts_ui = double(P_MACHINE_DATA.Ts_UIs);
if ~isfinite(Ts_ui) || Ts_ui <= 0
    Ts_ui = 0.05;
end

quat = double(bus_imu.quat(:));   % [w x y z]
gyro = double(bus_imu.gyro(:));   % [rad/s]
acc  = double(bus_imu.acc(:));    % [m/s^2]

if numel(quat) ~= 4 || numel(gyro) ~= 3 || numel(acc) ~= 3
    return;
end

if isempty(inited)
    windowSec = 1.5;
    Nbuf = max(20, ceil(windowSec / Ts_ui) + 3);
    Tbuf = zeros(1, Nbuf);
    Abuf = zeros(3, Nbuf);
    Gbuf = zeros(3, Nbuf);
    nsamp = uint32(0);
    kbuf  = uint32(0);
    frame_count = uint32(0);
    orient_div = uint32(6);   
    axis_div   = uint32(10);  
    last_xlim_update = 0.0;
    fig = figure('Name','IMU State','Position',[80 80 900 900], 'Tag','G1_IMUState');
    ax3 = subplot(3,1,1,'Parent',fig);
    title(ax3, {'IMU frame [quat]'; ' '});
    grid(ax3,'on');
    axis(ax3,'equal');
    xlim(ax3,[-1.1 1.1]);
    ylim(ax3,[-1.1 1.1]);
    zlim(ax3,[-1.1 1.1]);
    view(ax3,55,25);
    hold(ax3,'on');
    plot3(ax3,[-1.1 1.1],[0 0],[0 0],'k:');
    plot3(ax3,[0 0],[-1.1 1.1],[0 0],'k:');
    plot3(ax3,[0 0],[0 0],[-1.1 1.1],'k:');
    hX = plot3(ax3,[0 1],[0 0],[0 0],'LineWidth',3,'Color',[1 0 0]);
    hY = plot3(ax3,[0 0],[0 1],[0 0],'LineWidth',3,'Color',[0 0.5 0]);
    hZ = plot3(ax3,[0 0],[0 0],[0 1],'LineWidth',3,'Color',[0 0 1]);
    text(ax3, 1.675, 0.75, ' IMU frame [RPY]', ...
        'Units','normalized', ...
        'HorizontalAlignment','left', ...
        'FontWeight','bold', ...
        'FontSize',10, ...
        'Clipping','off');
    txtYPR = text(ax3, 1.675, 0.50, ...
        sprintf(['\\color[rgb]{1,0,0}Roll:  %+.2f°\\color{black}\n' ...
         '\\color[rgb]{0,0.5,0}Pitch: %+.2f°\\color{black}\n' ...
         '\\color[rgb]{0,0,1}Yaw:   %+.2f°\\color{black}'],0,0,0), ...
        'Units','normalized', ...
        'HorizontalAlignment','left', ...
        'Interpreter','tex', ...
        'FontWeight','bold', ...
        'BackgroundColor','none', ...
        'Color','k', ...
        'FontName','FixedWidth', ...
        'FontSize',11, ...
        'Clipping','off');
    hold(ax3,'off');
    set(ax3,'Position',[0.05 0.68 0.60 0.25]);

    axA = subplot(3,1,2,'Parent',fig);
    grid(axA,'on');
    title(axA,'Accelerometer');
    ylabel(axA,'Amplitude [m/s^2]');
    xlabel(axA,'Time [s]');
    xlim(axA,[-windowSec 0.0]);
    la1 = line(axA,0,0,'Color',[1 0 0]);
    la2 = line(axA,0,0,'Color',[0 0.5 0]);
    la3 = line(axA,0,0,'Color',[0 0 1]);
    legend(axA,{'ax','ay','az'},'Location','northeastoutside');

    axG = subplot(3,1,3,'Parent',fig);
    grid(axG,'on');
    title(axG,'Gyro');
    xlabel(axG,'Time [s]');
    ylabel(axG,'Amplitude [rad/s]');
    xlim(axG,[-windowSec 0.0]);
    lg1 = line(axG,0,0,'Color',[1 0 0]);
    lg2 = line(axG,0,0,'Color',[0 0.5 0]);
    lg3 = line(axG,0,0,'Color',[0 0 1]);
    legend(axG,{'gx','gy','gz'},'Location','northeastoutside');
    inited = true;
end

kbuf = kbuf + uint32(1);
if kbuf > uint32(Nbuf)
    kbuf = uint32(1);
end
k = double(kbuf);
if nsamp < uint32(Nbuf)
    nsamp = nsamp + uint32(1);
end
n = double(nsamp);
frame_count = frame_count + uint32(1);
if n == 1
    Tbuf(1,k) = 0.0;
else
    if k == 1
        kprev = Nbuf;
    else
        kprev = k - 1;
    end
    Tbuf(1,k) = Tbuf(1,kprev) + Ts_ui;
end
Abuf(:,k) = -acc(:);
Gbuf(:,k) = gyro(:);

if n < Nbuf
    tt = Tbuf(1,1:n);
    aa = Abuf(:,1:n);
    gg = Gbuf(:,1:n);
else
    if k < Nbuf
        ord = [k+1:Nbuf, 1:k];
    else
        ord = 1:Nbuf;
    end
    tt = Tbuf(ord);
    aa = Abuf(:,ord);
    gg = Gbuf(:,ord);
end

if ~isempty(tt)
    tt = tt - tt(end);
end

if mod(double(frame_count), double(orient_div)) == 0
    R  = quat2rotm_wxyz(quat(:)');
    ex = R(:,1);
    ey = R(:,2);
    ez = R(:,3);
    set(hX,'XData',[0 ex(1)],'YData',[0 ex(2)],'ZData',[0 ex(3)]);
    set(hY,'XData',[0 ey(1)],'YData',[0 ey(2)],'ZData',[0 ey(3)]);
    set(hZ,'XData',[0 ez(1)],'YData',[0 ez(2)],'ZData',[0 ez(3)]);
    [yaw,pitch,roll] = quat_to_ypr_zyx(quat(:)');
    set(txtYPR,'String',sprintf([ ...
        '\\color[rgb]{1,0,0}Roll:  %+.2f°\\color{black}\n' ...
        '\\color[rgb]{0,0.5,0}Pitch: %+.2f°\\color{black}\n' ...
        '\\color[rgb]{0,0,1}Yaw:   %+.2f°\\color{black}'], ...
        roll*180/pi, pitch*180/pi, yaw*180/pi));
end

set(la1,'XData',tt,'YData',aa(1,:));
set(la2,'XData',tt,'YData',aa(2,:));
set(la3,'XData',tt,'YData',aa(3,:));
set(lg1,'XData',tt,'YData',gg(1,:));
set(lg2,'XData',tt,'YData',gg(2,:));
set(lg3,'XData',tt,'YData',gg(3,:));

if mod(double(frame_count), double(axis_div)) == 0
    if abs(last_xlim_update - tt(end)) > 0.25 || frame_count == uint32(1)
        xlim(axA,[-windowSec 0.0]);
        xlim(axG,[-windowSec 0.0]);
        last_xlim_update = tt(end);
    end
    ylim_soft_fast(axA, aa);
    ylim_soft_fast(axG, gg);
end
drawnow limitrate nocallbacks;
end

function R = quat2rotm_wxyz(q)
w=q(1); x=q(2); y=q(3); z=q(4);
xx=x*x; yy=y*y; zz=z*z; wx=w*x; wy=w*y; wz=w*z; xy=x*y; xz=x*z; yz=y*z;
R=[1-2*(yy+zz)  2*(xy-wz)  2*(xz+wy);
   2*(xy+wz)  1-2*(xx+zz)  2*(yz-wx);
   2*(xz-wy)  2*(yz+wx)    1-2*(xx+yy)];
end

function [yaw,pitch,roll] = quat_to_ypr_zyx(q)
w=q(1); x=q(2); y=q(3); z=q(4);
yaw   = atan2(2*(w*z + x*y), 1 - 2*(y*y + z*z));
pitch = asin(max(-1,min(1, 2*(w*y - z*x))));
roll  = atan2(2*(w*x + y*z), 1 - 2*(x*x + y*y));
end

function ylim_soft_fast(ax, Y)
if isempty(Y)
    ylim(ax,[-1 1]);
    return;
end

m1 = max(abs(Y(1,:)));
m2 = max(abs(Y(2,:)));
m3 = max(abs(Y(3,:)));
v = max(1e-6, max([m1 m2 m3]));
ylim(ax,[-1.2*v, 1.2*v]);
end

== matlab function Sim2Real_variant_subsystem/SIM2REAL VARIANT SUBSYSTEM/ROS 2 SUBSYSTEM/ROS 2 SUBSYSTEM/JOINT COMMAND/BUILD motor_cmd BUS ==
  data: motor_cmd output Bus: SL_Bus_unitree_hg_MotorCmd; bus_tau_ref input Bus: bus_tau_ref; bus_pos_ref input Bus: bus_pos_ref; bus_vel_ref input Bus: bus_vel_ref; bus_kp_kd_dyn input Bus: bus_kp_kd_dyn
function motor_cmd = g1_build_motorcmd_vectors( ...
    bus_tau_ref, bus_pos_ref, bus_vel_ref, bus_kp_kd_dyn)
%#codegen

N     = int32(35);   
NBODY = int32(29);   
NLL = int32(6);   % left leg
NRL = int32(6);   % right leg
NW  = int32(3);   % waist
NLA = int32(7);   % left arm
NRA = int32(7);   % right arm

% tau refs
left_leg_tau_ref   = bus_tau_ref.left_leg_tau_ref;
right_leg_tau_ref  = bus_tau_ref.right_leg_tau_ref;
waist_tau_ref      = bus_tau_ref.waist_tau_ref;
left_arm_tau_ref   = bus_tau_ref.left_arm_tau_ref;
right_arm_tau_ref  = bus_tau_ref.right_arm_tau_ref;

% pos refs
left_leg_pos_ref   = bus_pos_ref.left_leg_pos_ref;
right_leg_pos_ref  = bus_pos_ref.right_leg_pos_ref;
waist_pos_ref      = bus_pos_ref.waist_pos_ref;
left_arm_pos_ref   = bus_pos_ref.left_arm_pos_ref;
right_arm_pos_ref  = bus_pos_ref.right_arm_pos_ref;

% vel refs
left_leg_vel_ref   = bus_vel_ref.left_leg_vel_ref;
right_leg_vel_ref  = bus_vel_ref.right_leg_vel_ref;
waist_vel_ref      = bus_vel_ref.waist_vel_ref;
left_arm_vel_ref   = bus_vel_ref.left_arm_vel_ref;
right_arm_vel_ref  = bus_vel_ref.right_arm_vel_ref;

% gains
left_leg_kp_kd     = bus_kp_kd_dyn.left_leg_kp_kd_dyn;
right_leg_kp_kd    = bus_kp_kd_dyn.right_leg_kp_kd_dyn;
waist_kp_kd        = bus_kp_kd_dyn.waist_kp_kd_dyn;
left_arm_kp_kd     = bus_kp_kd_dyn.left_arm_kp_kd_dyn;
right_arm_kp_kd    = bus_kp_kd_dyn.right_arm_kp_kd_dyn;

% Force shapes (column) and types
ll_q   = single(left_leg_pos_ref(:));   rl_q   = single(right_leg_pos_ref(:));
w_q    = single(waist_pos_ref(:));
la_q   = single(left_arm_pos_ref(:));   ra_q   = single(right_arm_pos_ref(:));

ll_dq  = single(left_leg_vel_ref(:));   rl_dq  = single(right_leg_vel_ref(:));
w_dq   = single(waist_vel_ref(:));
la_dq  = single(left_arm_vel_ref(:));   ra_dq  = single(right_arm_vel_ref(:));

ll_tau = single(left_leg_tau_ref(:));   rl_tau = single(right_leg_tau_ref(:));
w_tau  = single(waist_tau_ref(:));
la_tau = single(left_arm_tau_ref(:));   ra_tau = single(right_arm_tau_ref(:));

% Validate input sizes 
ok_ll = (int32(numel(ll_q))  == NLL) && (int32(numel(ll_dq))  == NLL) && (int32(numel(ll_tau))  == NLL);
ok_rl = (int32(numel(rl_q))  == NRL) && (int32(numel(rl_dq))  == NRL) && (int32(numel(rl_tau))  == NRL);
ok_w  = (int32(numel(w_q))   == NW ) && (int32(numel(w_dq))   == NW ) && (int32(numel(w_tau))   == NW );
ok_la = (int32(numel(la_q))  == NLA) && (int32(numel(la_dq))  == NLA) && (int32(numel(la_tau))  == NLA);
ok_ra = (int32(numel(ra_q))  == NRA) && (int32(numel(ra_dq))  == NRA) && (int32(numel(ra_tau))  == NRA);

% Gains: (6x2,6x2,3x2,7x2,7x2) -> 29 
ll_kp = get_col_or_default(left_leg_kp_kd,  1, NLL, single(60));  ll_kd = get_col_or_default(left_leg_kp_kd,  2, NLL, single(1));
rl_kp = get_col_or_default(right_leg_kp_kd, 1, NRL, single(60));  rl_kd = get_col_or_default(right_leg_kp_kd, 2, NRL, single(1));
w_kp  = get_col_or_default(waist_kp_kd,     1, NW,  single(40));  w_kd  = get_col_or_default(waist_kp_kd,     2, NW,  single(1));
la_kp = get_col_or_default(left_arm_kp_kd,  1, NLA, single(40));  la_kd = get_col_or_default(left_arm_kp_kd,  2, NLA, single(1));
ra_kp = get_col_or_default(right_arm_kp_kd, 1, NRA, single(40));  ra_kd = get_col_or_default(right_arm_kp_kd, 2, NRA, single(1));

% Concatenate BODY ONLY (29) 
q_body   = [fix_len(ll_q,NLL);  fix_len(rl_q,NRL);  fix_len(w_q,NW);  fix_len(la_q,NLA);  fix_len(ra_q,NRA)];
dq_body  = [fix_len(ll_dq,NLL); fix_len(rl_dq,NRL); fix_len(w_dq,NW); fix_len(la_dq,NLA); fix_len(ra_dq,NRA)];
tau_body = [fix_len(ll_tau,NLL);fix_len(rl_tau,NRL);fix_len(w_tau,NW); fix_len(la_tau,NLA);fix_len(ra_tau,NRA)];
kp_body  = [fix_len(ll_kp,NLL); fix_len(rl_kp,NRL); fix_len(w_kp,NW);  fix_len(la_kp,NLA); fix_len(ra_kp,NRA)];
kd_body  = [fix_len(ll_kd,NLL); fix_len(rl_kd,NRL); fix_len(w_kd,NW);  fix_len(la_kd,NLA); fix_len(ra_kd,NRA)];

M = int32(numel(q_body));
if M > NBODY
    M = NBODY; %#ok<NASGU>
end

motor_cmd = repmat( ...
    struct( ...
        'mode',    uint8(0), ...
        'q',       single(0), ...
        'dq',      single(0), ...
        'tau',     single(0), ...
        'kp',      single(0), ...
        'kd',      single(0), ...
        'reserve', uint32(0) ...
    ), ...
    double(N), 1);

% Left leg (1..6) 
if ok_ll
    for i = 1:6
        motor_cmd(i).mode    = uint8(1);
        motor_cmd(i).q       = q_body(i);
        motor_cmd(i).dq      = dq_body(i);
        motor_cmd(i).tau     = tau_body(i);
        motor_cmd(i).kp      = kp_body(i);
        motor_cmd(i).kd      = kd_body(i);
        motor_cmd(i).reserve = uint32(0);
    end
end

% Right leg (7..12)
if ok_rl
    for i = 7:12
        motor_cmd(i).mode    = uint8(1);
        motor_cmd(i).q       = q_body(i);
        motor_cmd(i).dq      = dq_body(i);
        motor_cmd(i).tau     = tau_body(i);
        motor_cmd(i).kp      = kp_body(i);
        motor_cmd(i).kd      = kd_body(i);
        motor_cmd(i).reserve = uint32(0);
    end
end

% Waist (13..15) 
if ok_w
    for i = 13:15
        motor_cmd(i).mode    = uint8(1);
        motor_cmd(i).q       = q_body(i);
        motor_cmd(i).dq      = dq_body(i);
        motor_cmd(i).tau     = tau_body(i);
        motor_cmd(i).kp      = kp_body(i);
        motor_cmd(i).kd      = kd_body(i);
        motor_cmd(i).reserve = uint32(0);
    end
end

% Left arm (16..22)
if ok_la
    for i = 16:22
        motor_cmd(i).mode    = uint8(1);
        motor_cmd(i).q       = q_body(i);
        motor_cmd(i).dq      = dq_body(i);
        motor_cmd(i).tau     = tau_body(i);
        motor_cmd(i).kp      = kp_body(i);
        motor_cmd(i).kd      = kd_body(i);
        motor_cmd(i).reserve = uint32(0);
    end
end

% Right arm (23..29)
if ok_ra
    for i = 23:29
        motor_cmd(i).mode    = uint8(1);
        motor_cmd(i).q       = q_body(i);
        motor_cmd(i).dq      = dq_body(i);
        motor_cmd(i).tau     = tau_body(i);
        motor_cmd(i).kp      = kp_body(i);
        motor_cmd(i).kd      = kd_body(i);
        motor_cmd(i).reserve = uint32(0);
    end
end

motor_cmd(14).mode = uint8(0);  % waist roll  (index 13)
motor_cmd(15).mode = uint8(0);  % waist pitch (index 14)

end

function y = fix_len(x, L)
y = zeros(double(L),1,'single');
n = int32(numel(x));
m = n;
if m > L
    m = L;
end
if m > 0
    y(1:double(m)) = x(1:double(m));
end
end

function v = get_col_or_default(M, col, L, default_val)
v = default_val * ones(double(L),1,'single');
if ~isempty(M) && (size(M,2) >= col)
    tmp = single(M(:,col));
    n = int32(numel(tmp));
    m = n;
    if m > L
        m = L;
    end
    if m > 0
        v(1:double(m)) = tmp(1:double(m));
    end
end
end

== matlab function Sim2Real_variant_subsystem/SIM2REAL VARIANT SUBSYSTEM/ROS 2 SUBSYSTEM/ROS 2 SUBSYSTEM/JOINT COMMAND/BUILD CRC ==
  data: cmd_in input; crc_out output
function crc_out = g1_crc_lowcmd_optionA(cmd_in)
%#codegen

N = 35;          
PACK_LEN = 1004; 
cmd = cmd_in;
cmd.crc = uint32(0);
pack = zeros(PACK_LEN, 1, 'uint8');
k = int32(1);

% ---- '<2B2x' ----
pack(k) = uint8(cmd.mode_pr);      k = k + 1;
pack(k) = uint8(cmd.mode_machine); k = k + 1;
pack(k) = uint8(0);                k = k + 1;
pack(k) = uint8(0);                k = k + 1;

% ---- 'B3x5fI' * 35 ----
for i = 1:N
    pack(k) = uint8(cmd.motor_cmd(i).mode); k = k + 1;
    % 3x padding
    pack(k) = uint8(0); k = k + 1;
    pack(k) = uint8(0); k = k + 1;
    pack(k) = uint8(0); k = k + 1;
    [pack,k] = write_f32(pack,k, single(cmd.motor_cmd(i).q));
    [pack,k] = write_f32(pack,k, single(cmd.motor_cmd(i).dq));
    [pack,k] = write_f32(pack,k, single(cmd.motor_cmd(i).tau));
    [pack,k] = write_f32(pack,k, single(cmd.motor_cmd(i).kp));
    [pack,k] = write_f32(pack,k, single(cmd.motor_cmd(i).kd));
    [pack,k] = write_u32(pack,k, uint32(cmd.motor_cmd(i).reserve));
end

% ---- '5I' => reserve[4] + crc placeholder ----
for r = 1:4
    [pack,k] = write_u32(pack,k, uint32(cmd.reserve(r)));
end
[pack,k] = write_u32(pack,k, uint32(0)); % crc placeholder

if k ~= int32(PACK_LEN + 1)
    crc_out = uint32(0);
    return;
end

WORDS = 250; % (1004/4) - 1
words = zeros(WORDS,1,'uint32');

for i = 1:WORDS
    base = (i-1)*4;
    b0 = uint32(pack(base+1));
    b1 = bitshift(uint32(pack(base+2)), 8);
    b2 = bitshift(uint32(pack(base+3)), 16);
    b3 = bitshift(uint32(pack(base+4)), 24);
    words(i) = bitor(bitor(b0,b1), bitor(b2,b3));
end

crc_out = crc32_core_unitree(words);
end

function [buf,k] = write_f32(buf,k,v)
b = typecast(single(v), 'uint8');
buf(k:k+3) = b(:);
k = k + 4;
end

function [buf,k] = write_u32(buf,k,v)
b = typecast(uint32(v), 'uint8');
buf(k:k+3) = b(:);
k = k + 4;
end

function crc = crc32_core_unitree(data)
crc  = uint32(4294967295);     % 0xFFFFFFFF
poly = uint32(79764919);       % 0x04C11DB7
MSB  = uint32(2147483648);     % 1<<31

for i = 1:numel(data)
    current = uint32(data(i));
    bit = MSB;
    for b = 1:32
        if bitand(crc, MSB) ~= 0
            crc = bitxor(bitshift(crc,1), poly);
        else
            crc = bitshift(crc,1);
        end
        if bitand(current, bit) ~= 0
            crc = bitxor(crc, poly);
        end
        bit = bitshift(bit, -1);
    end
end
end
